simulink model "csp_planning"  (R2023a)
settings: configuration reference "config" (kept outside this file)
undefined symbols (not defined in the file): DiscIntNeverNeededParam
settings Model: DataDictionary=model_config.sldd  Creator=huangcheng  LastModifiedBy=Administrator
settings ConfigSetRef: SourceName=config

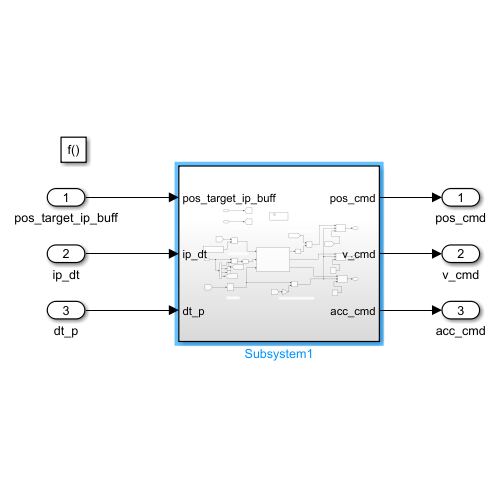
[thumbnail: Simulink's stored preview of the top-level diagram]
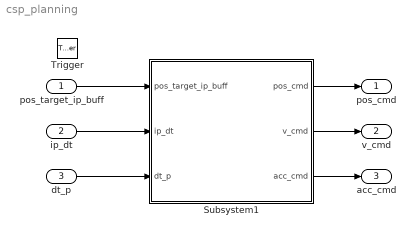
== system csp_planning ==
  pos_target_ip_buff : Inport
  ip_dt : Inport  Port=2
  dt_p : Inport  Port=3
  Trigger : TriggerPort  TriggerType=function-call  VariantControl=(inherit)  PortDimensions=1
  Subsystem1 : Subsystem  SystemSampleTime=10e-5
  pos_cmd : Outport
  v_cmd : Outport  Port=2
  acc_cmd : Outport  Port=3
  wires:
  dt_p/1 -> Subsystem1/3(dt_p)
  pos_target_ip_buff/1 -> Subsystem1/1(pos_target_ip_buff)
  ip_dt/1 -> Subsystem1/2(ip_dt)
  Subsystem1/3(acc_cmd) -> acc_cmd/1
  Subsystem1/1(pos_cmd) -> pos_cmd/1
  Subsystem1/2(v_cmd) -> v_cmd/1

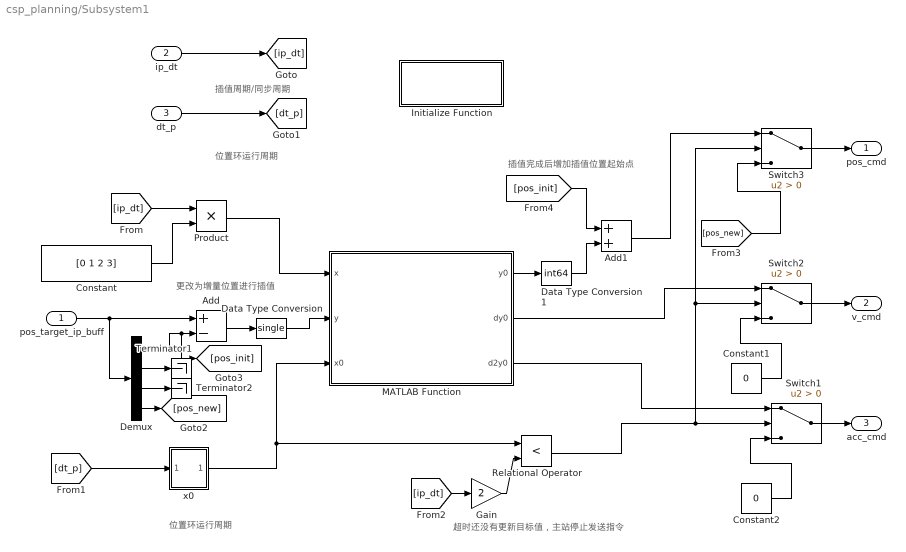
== system csp_planning/Subsystem1 ==
  note: 更改为增量位置进行插值
  note: 位置环运行周期
  note: 插值周期/同步周期
  note: 位置环运行周期
  note: 超时还没有更新目标值，主站停止发送指令
  note: 插值完成后增加插值位置起始点
  pos_target_ip_buff : Inport  OutDataTypeStr=int64  PortDimensions=4
  ip_dt : Inport  Port=2
  dt_p : Inport  Port=3
  Add : Sum  Inputs=+-
  Add1 : Sum
  Constant : Constant  Value=[0 1 2 3]  OutDataTypeStr=single
  Constant1 : Constant  Value=0  OutDataTypeStr=single
  Constant2 : Constant  Value=0  OutDataTypeStr=single
  Data Type Conversion : DataTypeConversion  OutDataTypeStr=single  SaturateOnIntegerOverflow=off  RndMeth=Floor
  Data Type Conversion1 : DataTypeConversion  OutDataTypeStr=int64  SaturateOnIntegerOverflow=off  RndMeth=Floor
  Demux : Demux
  Gain : Gain  Gain=2
  Initialize Function : Subsystem  TreatAsAtomicUnit=on
  MATLAB Function : MATLAB Function  SystemSampleTime=10e-5
  Product : Product
  Relational Operator : RelationalOperator  Operator=<  OutDataTypeStr=boolean  RndMeth=Simplest  InputSameDT=off
  Switch1 : Switch  Criteria=u2 > Threshold  SaturateOnIntegerOverflow=off  InputSameDT=off
  Switch2 : Switch  Criteria=u2 > Threshold  SaturateOnIntegerOverflow=off  InputSameDT=off
  Switch3 : Switch  Criteria=u2 > Threshold  SaturateOnIntegerOverflow=off  InputSameDT=off
  Terminator1 : Terminator
  Terminator2 : Terminator
  x0 : Subsystem
  pos_cmd : Outport
  v_cmd : Outport  Port=2
  acc_cmd : Outport  Port=3
  wires:
  Constant/1 -> Product/2
  [ip_dt] -> Product/1
  ip_dt/1 -> [ip_dt]
  dt_p/1 -> [dt_p]
  Product/1 -> MATLAB Function/1(x)
  pos_target_ip_buff/1 -> Add/1, Demux/1
  [dt_p] -> x0/1(In1)
  [ip_dt] -> Gain/1
  Gain/1 -> Relational Operator/2
  x0/1(Out1) -> MATLAB Function/3(x0), Relational Operator/1
  Constant2/1 -> Switch1/3
  Switch1/1 -> acc_cmd/1
  MATLAB Function/3(d2y0) -> Switch1/1
  MATLAB Function/2(dy0) -> Switch2/1
  Constant1/1 -> Switch2/3
  Switch2/1 -> v_cmd/1
  [pos_new] -> Switch3/3
  Relational Operator/1 -> Switch2/2, Switch3/2, Switch1/2
  Switch3/1 -> pos_cmd/1
  Demux/1 -> [pos_init], Add/2
  Demux/2 -> Terminator1/1
  Demux/3 -> Terminator2/1
  Demux/4 -> [pos_new]
  Add/1 -> Data Type Conversion/1
  Data Type Conversion/1 -> MATLAB Function/2(y)
  [pos_init] -> Add1/1
  Add1/1 -> Switch3/1
  MATLAB Function/1(y0) -> Data Type Conversion1/1
  Data Type Conversion1/1 -> Add1/2

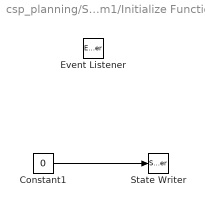
== system csp_planning/Subsystem1/Initialize Function ==
  Constant1 : Constant  Value=0  OutDataTypeStr=single
  Event Listener : EventListener  DisableCoverage=on  EventName=reset
  State Writer : StateWriter  StateOwnerBlock=../../x0/Discrete-Time Integrator  StateName=x0_sum
  wires:
  Constant1/1 -> State Writer/1

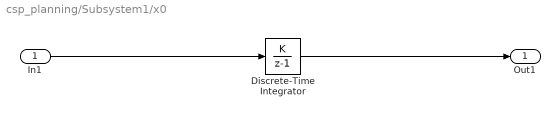
== system csp_planning/Subsystem1/x0 ==
  In1 : Inport
  Discrete-Time Integrator : DiscreteIntegrator  IntegratorMethod=Accumulation: Forward Euler  SampleTime=-1  StateName=x0_sum  ICPrevOutput=DiscIntNeverNeededParam  ICPrevScaledInput=DiscIntNeverNeededParam
  Out1 : Outport
  wires:
  In1/1 -> Discrete-Time Integrator/1
  Discrete-Time Integrator/1 -> Out1/1

== matlab function csp_planning/Subsystem1/MATLAB Function ==
  data: x input; y input; y0 output; x0 input; dy0 output; d2y0 output
function [y0, dy0, d2y0]  = interpolateSignal(x,y,x0)
 
% 可选插值方法pchip、 makima 、spline一阶导数和二阶导数
    % 输入:
    %   pp - 返回的分段多项式结构
    %   x0 - 要计算的点（可以是向量）
    % 输出:
    %   y0  - 函数值
    %   dy0 - 一阶导数
    %   d2y0 - 二阶导数

    pp = makima(x, y);

    % 1. 计算函数值
    y0 = ppval(pp, x0);
    
     % 方法二：手动从系数计算
    breaks = pp.breaks;
    coefs = pp.coefs;

    %x0必须始终在插值第一段

    c = coefs(1, :);  % 系数为 [a, b, c, d]，对应 (x-break)^3, (x-break)^2, (x-break)^1, 常数项
    t = x0 - breaks(1);
    % 一阶导数
    dy0 = 3*c(1)*t^2 + 2*c(2)*t + c(3);
    % 二阶导数
    d2y0 = 6*c(1)*t + 2*c(2);

end
